simulink model "rocket_6dof_simulation"  (R2026b)
settings: Solver=ode4  StopTime=sim_stopTime  FixedStep=sim_fixedStep
undefined symbols (not defined in the file): aero_refLength, CG, chute_attachBody, chute_CdS, chute_inflateTau, chute_riserLength, Cl_delta, Cl_p, Cm_a, Cm_q, Cn_b, Cn_r, command_stepTime, controller_inner_Kp, controller_outer_Kp, controller_outer_maxRateCmd, CP, Cx_0, Cy_0, Cy_b, Cz_0, Cz_a, environment_g, environment_wind, fin_actuatorTau, fin_maxDeflection, fin_maxRate, Fth, initial_euler, initial_position, initial_pqr, initial_velocityBody, Isp, propulsion_cutoffTime, rocket_cg0, rocket_mass0, rocket_massDry, sensor_attitudeTau, sensor_gyroTau
libraries: aerolibasang x3, simulink x3, aerolibatmos2 x1, shared6dof x1
settings Model: Creator=kiwamoto  LastModifiedBy=kiwamoto

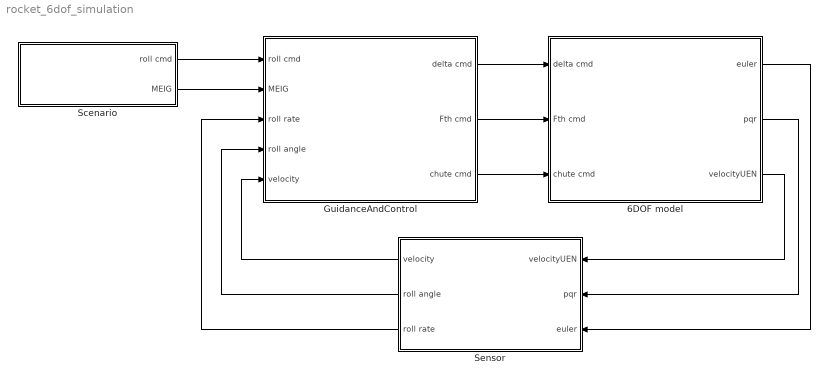
== system rocket_6dof_simulation ==
  6DOF model : Subsystem
  GuidanceAndControl : Subsystem
  Scenario : Subsystem
  Sensor : Subsystem
  wires:
  Scenario/1(roll cmd) -> GuidanceAndControl/1(roll cmd)
  GuidanceAndControl/1(delta cmd) -> 6DOF model/1(delta cmd)
  6DOF model/2(pqr) -> Sensor/2(pqr)
  6DOF model/1(euler) -> Sensor/3(euler)
  Sensor/2(roll angle) -> GuidanceAndControl/4(roll angle)
  Sensor/3(roll rate) -> GuidanceAndControl/3(roll rate)
  GuidanceAndControl/2(Fth cmd) -> 6DOF model/2(Fth cmd)
  Scenario/2(MEIG) -> GuidanceAndControl/2(MEIG)
  6DOF model/3(velocityUEN) -> Sensor/1(velocityUEN)
  GuidanceAndControl/3(chute cmd) -> 6DOF model/3(chute cmd)
  Sensor/1(velocity) -> GuidanceAndControl/5(velocity)

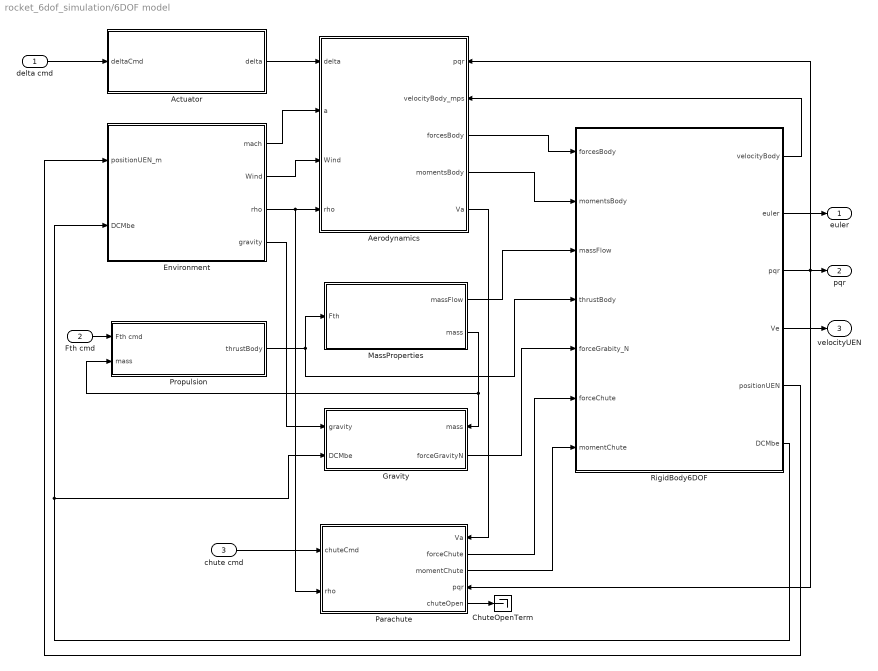
== system rocket_6dof_simulation/6DOF model ==
  delta cmd : Inport
  Fth cmd : Inport  Port=2
  chute cmd : Inport  Port=3
  Actuator : Subsystem
  Aerodynamics : Subsystem
      settings: PortSchema="{\"entries\":[{\"content\":{\"sides\":[{\"content\":{\"connectorIds\":[\"In1\",\"In2\",\"In3\",\"In4\"]},\"type\":\"ConnectorPlacement.EquallySpacedRectSide\",\"uuid\":\"af4c3f3a-b32b-4852-bfef-16d4a55bc85d\"},{\"content\":{\"connectorIds\":[\"In5\",\"In6\",\"Out1\",\"Out2\",\"Out3\"],\"side\":\"RIGHT\"},\"type\":\"ConnectorPlacement.EquallySpacedRectSide\",\"uuid\":\"ec426dca-c226-4b80-bf23-7134222deebc\"},{\"content\":{\"side\":\"TOP\"},\"type\":\"ConnectorPlacement.EquallySpacedRectSide\",\"uuid\":\"6bf281c2-d4c8-4f95-a415-10d5fcb30e4a\"}]},\"type\":\"ConnectorPlacement.EquallySpacedConnector\",\"uuid\":\"b5802e10-4233-47a2-b97a-a8820a58bc73\"}],\"packageUris\":[\"http://schema.mathworks.com/mf0/Connector/R2020b\"],\"version\":\"1.0\"}"
  ChuteOpenTerm : Terminator
  Environment : Subsystem
  Gravity : Subsystem
      settings: PortSchema="{\"entries\":[{\"content\":{\"sides\":[{\"content\":{\"connectorIds\":[\"In1\",\"In2\"]},\"type\":\"ConnectorPlacement.EquallySpacedRectSide\",\"uuid\":\"58b48f2a-cd32-4d34-a1ae-ee392d32123b\"},{\"content\":{\"connectorIds\":[\"In3\",\"Out1\"],\"side\":\"RIGHT\"},\"type\":\"ConnectorPlacement.EquallySpacedRectSide\",\"uuid\":\"b043d20d-e312-4365-ac79-6f9f081e3e75\"},{\"content\":{\"side\":\"TOP\"},\"type\":\"ConnectorPlacement.EquallySpacedRectSide\",\"uuid\":\"7786ccd6-2d55-46d0-949f-224f2e6bbbde\"}]},\"type\":\"ConnectorPlacement.EquallySpacedConnector\",\"uuid\":\"7e0c739f-134e-4285-a217-42daec375290\"}],\"packageUris\":[\"http://schema.mathworks.com/mf0/Connector/R2020b\"],\"version\":\"1.0\"}"
  MassProperties : Subsystem
  Parachute : Subsystem
      settings: PortSchema="{\"entries\":[{\"content\":{\"sides\":[{\"content\":{\"connectorIds\":[\"In1\",\"In2\"]},\"type\":\"ConnectorPlacement.EquallySpacedRectSide\",\"uuid\":\"ab562e91-55ed-4f52-87b8-211519146483\"},{\"content\":{\"connectorIds\":[\"In3\",\"Out1\",\"Out2\",\"In4\",\"Out3\"],\"side\":\"RIGHT\"},\"type\":\"ConnectorPlacement.EquallySpacedRectSide\",\"uuid\":\"d1f95e4e-60be-4e36-afec-0b6bd2c0f004\"},{\"content\":{\"side\":\"TOP\"},\"type\":\"ConnectorPlacement.EquallySpacedRectSide\",\"uuid\":\"dc12724e-5caf-4014-9240-a32a59dbf896\"}]},\"type\":\"ConnectorPlacement.EquallySpacedConnector\",\"uuid\":\"e57dcaa1-2a9c-4da6-8406-b82df234227e\"}],\"packageUris\":[\"http://schema.mathworks.com/mf0/Connector/R2020b\"],\"version\":\"1.0\"}"
  Propulsion : Subsystem
  RigidBody6DOF : Subsystem
  euler : Outport
  pqr : Outport  Port=2
  velocityUEN : Outport  Port=3
  wires:
  RigidBody6DOF/3(pqr) -> Parachute/4(pqr), pqr/1, Aerodynamics/5(pqr)
  MassProperties/2(mass) -> Propulsion/2(mass), Gravity/3(mass)
  RigidBody6DOF/1(velocityBody) -> Aerodynamics/6(velocityBody_mps)
  Actuator/1(delta) -> Aerodynamics/1(delta)
  Aerodynamics/2(momentsBody) -> RigidBody6DOF/2(momentsBody)
  Aerodynamics/1(forcesBody) -> RigidBody6DOF/1(forcesBody)
  Propulsion/1(thrustBody) -> RigidBody6DOF/4(thrustBody), MassProperties/1(Fth)
  delta cmd/1 -> Actuator/1(deltaCmd)
  RigidBody6DOF/2(euler) -> euler/1
  Environment/3(rho) -> Aerodynamics/4(rho), Parachute/2(rho)
  Environment/4(gravity) -> Gravity/1(gravity)
  RigidBody6DOF/6(DCMbe) -> Gravity/2(DCMbe), Environment/2(DCMbe)
  Gravity/1(forceGravityN) -> RigidBody6DOF/5(forceGrabity_N)
  Environment/2(Wind) -> Aerodynamics/3(Wind)
  Environment/1(mach) -> Aerodynamics/2(a)
  RigidBody6DOF/5(positionUEN) -> Environment/1(positionUEN_m)
  Fth cmd/1 -> Propulsion/1(Fth cmd)
  MassProperties/1(massFlow) -> RigidBody6DOF/3(massFlow)
  chute cmd/1 -> Parachute/1(chuteCmd)
  Aerodynamics/3(Va) -> Parachute/3(Va)
  Parachute/3(chuteOpen) -> ChuteOpenTerm/1
  Parachute/1(forceChute) -> RigidBody6DOF/6(forceChute)
  Parachute/2(momentChute) -> RigidBody6DOF/7(momentChute)
  RigidBody6DOF/4(Ve) -> velocityUEN/1

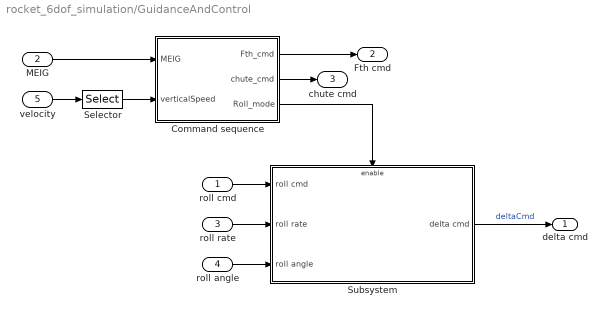
== system rocket_6dof_simulation/GuidanceAndControl ==
  roll cmd : Inport
  MEIG : Inport  Port=2
  roll rate : Inport  Port=3
  roll angle : Inport  Port=4
  velocity : Inport  Port=5
  Command sequence : Stateflow chart  TreatAsAtomicUnit=on
      settings: PortSchema="{\"entries\":[{\"content\":{\"sides\":[{\"content\":{\"connectorIds\":[\"In1\",\"In2\"]},\"type\":\"ConnectorPlacement.EquallySpacedRectSide\",\"uuid\":\"95c67331-47e3-44af-bd01-16a94959fc95\"},{\"content\":{\"connectorIds\":[\"Out1\",\"Out3\",\"Out2\"],\"side\":\"RIGHT\"},\"type\":\"ConnectorPlacement.EquallySpacedRectSide\",\"uuid\":\"42b891d2-3784-42c1-a532-d1c942f19e32\"},{\"content\":{\"side\":\"TOP\"},\"type\":\"ConnectorPlacement.EquallySpacedRectSide\",\"uuid\":\"6230014a-0262-43f4-a38a-a38e632e5bb9\"}]},\"type\":\"ConnectorPlacement.EquallySpacedConnector\",\"uuid\":\"a3f4a931-66e7-452b-9163-9591630e354f\"}],\"packageUris\":[\"http://schema.mathworks.com/mf0/Connector/R2020b\"],\"version\":\"1.0\"}"
  Selector : Selector  InputPortWidth=3  IndexOptions=Index vector (dialog)  Indices=1  OutputSizes=1  RuntimeRangeChecks=off
  Subsystem : Subsystem
  delta cmd : Outport
  Fth cmd : Outport  Port=2
  chute cmd : Outport  Port=3
  wires:
  Command sequence/1(Fth_cmd) -> Fth cmd/1
  MEIG/1 -> Command sequence/1(MEIG)
  roll cmd/1 -> Subsystem/1(roll cmd)
  roll rate/1 -> Subsystem/2(roll rate)
  roll angle/1 -> Subsystem/3(roll angle)
  Subsystem/1(delta cmd) -> delta cmd/1  "deltaCmd"
  Command sequence/2(Roll_mode) -> Subsystem/Enable
  velocity/1 -> Selector/1
  Command sequence/3(chute_cmd) -> chute cmd/1
  Selector/1 -> Command sequence/2(verticalSpeed)

== system rocket_6dof_simulation/Scenario ==
  On : Constant
  RollCommandStep : Step  Time=command_stepTime  FinalValue=command_rollStep  SampleTime=0
  roll cmd : Outport
  MEIG : Outport  Port=2
  wires:
  RollCommandStep/1 -> roll cmd/1  "phiCmd"
  On/1 -> MEIG/1

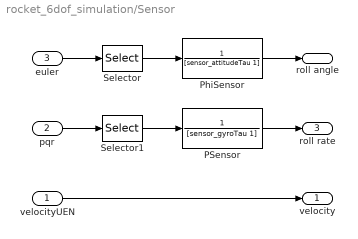
== system rocket_6dof_simulation/Sensor ==
  velocityUEN : Inport
  pqr : Inport  Port=2
  euler : Inport  Port=3
  PSensor : TransferFcn  Denominator=[sensor_gyroTau 1]
  PhiSensor : TransferFcn  Denominator=[sensor_attitudeTau 1]
  Selector : Selector  InputPortWidth=3  IndexOptions=Index vector (dialog)  Indices=1  OutputSizes=1  RuntimeRangeChecks=off
  Selector1 : Selector  InputPortWidth=3  IndexOptions=Index vector (dialog)  Indices=1  OutputSizes=1  RuntimeRangeChecks=off
  velocity : Outport
  roll angle : Outport  Port=2
  roll rate : Outport  Port=3
  wires:
  pqr/1 -> Selector1/1
  PhiSensor/1 -> roll angle/1
  Selector/1 -> PhiSensor/1
  Selector1/1 -> PSensor/1
  euler/1 -> Selector/1
  PSensor/1 -> roll rate/1
  velocityUEN/1 -> velocity/1

== system rocket_6dof_simulation/6DOF model/Actuator ==
  deltaCmd : Inport
  FinActuator : TransferFcn  Denominator=[fin_actuatorTau 1]
  FinRateLimiter : RateLimiter  RisingSlewLimit=fin_maxRate  FallingSlewLimit=-fin_maxRate  SampleTimeMode=inherited
  FinSaturation : Saturate  UpperLimit=fin_maxDeflection  LowerLimit=-fin_maxDeflection
  delta : Outport
  wires:
  deltaCmd/1 -> FinRateLimiter/1
  FinRateLimiter/1 -> FinSaturation/1
  FinSaturation/1 -> FinActuator/1
  FinActuator/1 -> delta/1  "delta"

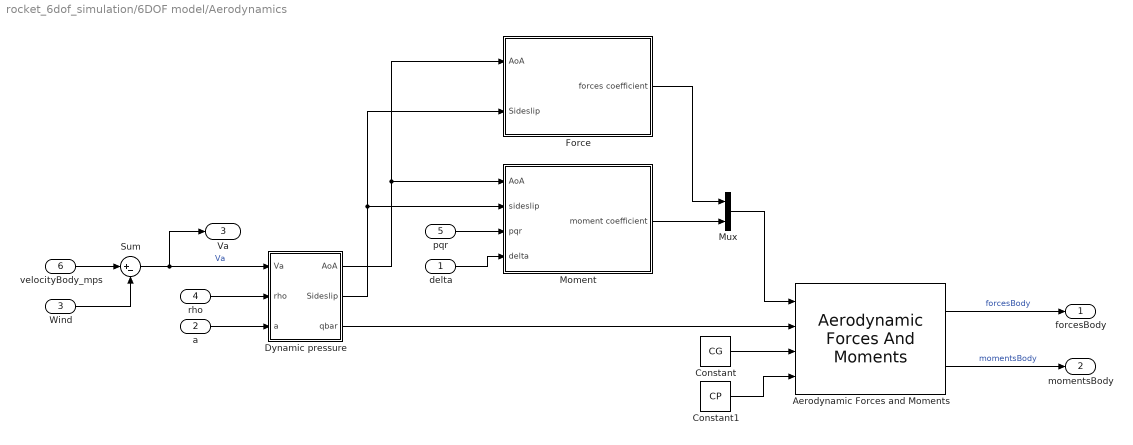
== system rocket_6dof_simulation/6DOF model/Aerodynamics ==
  delta : Inport
  a : Inport  Port=2
  Wind : Inport  Port=3
  rho : Inport  Port=4
  pqr : Inport  Port=5
  velocityBody_mps : Inport  Port=6
  "Aerodynamic Forces and Moments " : AerodynamicForcesAndMoments  S=aero_refArea  b=aero_refLength  cbar=aero_refLength
  Constant : Constant  Value=CG
  Constant1 : Constant  Value=CP
  Dynamic pressure : Subsystem
  Force : Subsystem
  Moment : Subsystem
  Mux : Mux  Inputs=2
  Sum : Sum  Inputs=|+-
  forcesBody : Outport
  momentsBody : Outport  Port=2
  Va : Outport  Port=3
  wires:
  delta/1 -> Moment/4(delta)
  rho/1 -> Dynamic pressure/2(rho)
  velocityBody_mps/1 -> Sum/1
  Wind/1 -> Sum/2
  Sum/1 -> Dynamic pressure/1(Va), Va/1  "Va"
  a/1 -> Dynamic pressure/3(a)
  "Aerodynamic Forces and Moments "/1 -> forcesBody/1  "forcesBody"
  "Aerodynamic Forces and Moments "/2 -> momentsBody/1  "momentsBody"
  Dynamic pressure/3(qbar) -> "Aerodynamic Forces and Moments "/2
  pqr/1 -> Moment/3(pqr)
  Mux/1 -> "Aerodynamic Forces and Moments "/1
  Moment/1(moment coefficient) -> Mux/2
  Force/1(forces coefficient) -> Mux/1
  Dynamic pressure/1(AoA) -> Force/1(AoA), Moment/1(AoA)
  Dynamic pressure/2(Sideslip) -> Force/2(Sideslip), Moment/2(sideslip)
  Constant/1 -> "Aerodynamic Forces and Moments "/3
  Constant1/1 -> "Aerodynamic Forces and Moments "/4

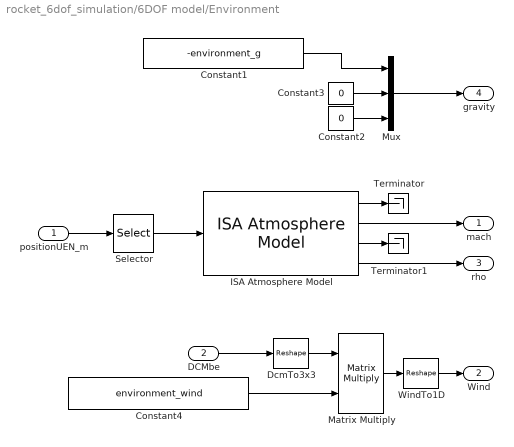
== system rocket_6dof_simulation/6DOF model/Environment ==
  positionUEN_m : Inport
  DCMbe : Inport  Port=2
  Constant1 : Constant  Value=-environment_g
  Constant2 : Constant  Value=0
  Constant3 : Constant  Value=0
  Constant4 : Constant  Value=environment_wind
  DcmTo3x3 : Reshape  OutputDimensionality=Customize  OutputDimensions=[3 3]
  ISA Atmosphere Model : aerolibatmos2/ISA Atmosphere Model  useExtended=off  action=None  custom=off  viscosityOut=off  g=9.80665  gamma=1.4  R=287.0531  L=0.0065  h_trop=11000  h_strat=20000  rho0=1.225  P0=101325  T0=288.15  h0=0  S=110.4  Tref=273.15  muref=1.716e-5
  Matrix Multiply : Product  Multiplication=Matrix(*)
  Mux : Mux  Inputs=3
  Selector : Selector  InputPortWidth=3  IndexOptions=Index vector (dialog)  Indices=1  OutputSizes=1  RuntimeRangeChecks=off
  Terminator : Terminator
  Terminator1 : Terminator
  WindTo1D : Reshape
  mach : Outport
  Wind : Outport  Port=2
  rho : Outport  Port=3
  gravity : Outport  Port=4
  wires:
  ISA Atmosphere Model/4 -> rho/1
  Mux/1 -> gravity/1
  Constant2/1 -> Mux/3
  Constant3/1 -> Mux/2
  Constant1/1 -> Mux/1
  Constant4/1 -> Matrix Multiply/2
  ISA Atmosphere Model/2 -> mach/1
  ISA Atmosphere Model/1 -> Terminator/1
  ISA Atmosphere Model/3 -> Terminator1/1
  positionUEN_m/1 -> Selector/1
  Selector/1 -> ISA Atmosphere Model/1
  Matrix Multiply/1 -> WindTo1D/1
  WindTo1D/1 -> Wind/1
  DCMbe/1 -> DcmTo3x3/1
  DcmTo3x3/1 -> Matrix Multiply/1

== system rocket_6dof_simulation/6DOF model/Gravity ==
  gravity : Inport
  DCMbe : Inport  Port=2
  mass : Inport  Port=3
  DcmTo3x3 : Reshape  OutputDimensionality=Customize  OutputDimensions=[3 3]
  GravityTo1D : Reshape
  Product : Product  Multiplication=Matrix(*)
  Product1 : Product
  forceGravityN : Outport
  wires:
  Product/1 -> GravityTo1D/1
  GravityTo1D/1 -> forceGravityN/1
  DCMbe/1 -> DcmTo3x3/1
  DcmTo3x3/1 -> Product/1
  gravity/1 -> Product1/1
  mass/1 -> Product1/2
  Product1/1 -> Product/2

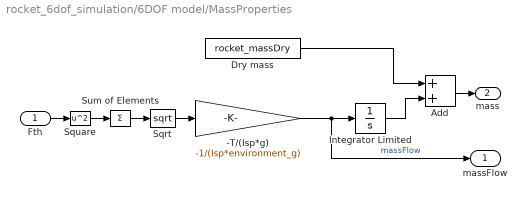
== system rocket_6dof_simulation/6DOF model/MassProperties ==
  Fth : Inport
  -T/(Isp*g) : Gain  Gain=-1/(Isp*environment_g)
  Add : Sum
  Dry mass : Constant  Value=rocket_massDry
  Integrator Limited : Integrator  InitialCondition=rocket_mass0 - rocket_massDry  LimitOutput=on  UpperSaturationLimit=rocket_mass0 - rocket_massDry  LowerSaturationLimit=0
  Sqrt : Sqrt
  Square : Math  Operator=square
  Sum of Elements : Sum  Inputs=+
  massFlow : Outport
  mass : Outport  Port=2
  wires:
  Dry mass/1 -> Add/1
  Integrator Limited/1 -> Add/2
  Add/1 -> mass/1
  -T/(Isp*g)/1 -> Integrator Limited/1, massFlow/1  "massFlow"
  Fth/1 -> Square/1
  Square/1 -> Sum of Elements/1
  Sum of Elements/1 -> Sqrt/1
  Sqrt/1 -> -T/(Isp*g)/1

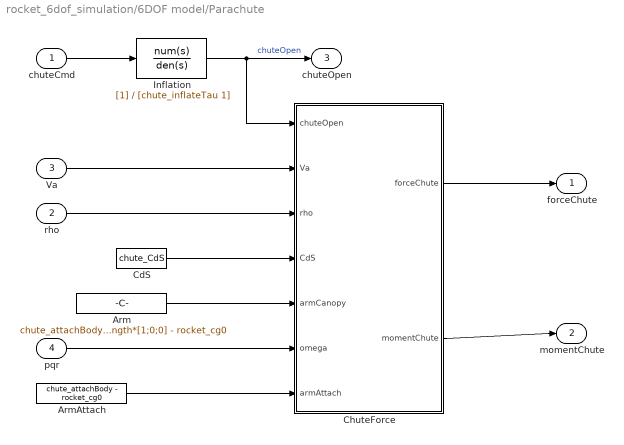
== system rocket_6dof_simulation/6DOF model/Parachute ==
  chuteCmd : Inport
  rho : Inport  Port=2
  Va : Inport  Port=3
  pqr : Inport  Port=4
  Arm : Constant  Value=chute_attachBody + chute_riserLength*[1;0;0] - rocket_cg0
  ArmAttach : Constant  Value=chute_attachBody - rocket_cg0
  CdS : Constant  Value=chute_CdS
  ChuteForce : MATLAB Function  TreatAsAtomicUnit=on
  Inflation : TransferFcn  Denominator=[chute_inflateTau 1]
  forceChute : Outport
  momentChute : Outport  Port=2
  chuteOpen : Outport  Port=3
  wires:
  chuteCmd/1 -> Inflation/1
  Inflation/1 -> ChuteForce/1(chuteOpen), chuteOpen/1  "chuteOpen"
  Va/1 -> ChuteForce/2(Va)
  rho/1 -> ChuteForce/3(rho)
  CdS/1 -> ChuteForce/4(CdS)
  Arm/1 -> ChuteForce/5(armCanopy)
  ChuteForce/1(forceChute) -> forceChute/1
  ChuteForce/2(momentChute) -> momentChute/1
  pqr/1 -> ChuteForce/6(omega)
  ArmAttach/1 -> ChuteForce/7(armAttach)

== system rocket_6dof_simulation/6DOF model/Propulsion ==
  Fth cmd : Inport
  mass : Inport  Port=2
  Compare To Constant : simulink/Logic and Bit Operations/Compare To Constant  relop=>  const=rocket_massDry  OutDataTypeStr=boolean
  Product : Product
  ThrustMux : Mux  Inputs=3
  ZeroY : Constant  Value=0
  ZeroZ : Constant  Value=0
  burn delay : TransferFcn  Denominator=[0.05 1]
  thrustBody : Outport
  wires:
  ZeroY/1 -> ThrustMux/2
  ZeroZ/1 -> ThrustMux/3
  ThrustMux/1 -> thrustBody/1
  Fth cmd/1 -> burn delay/1
  mass/1 -> Compare To Constant/1
  Product/1 -> ThrustMux/1  "thrust"
  Compare To Constant/1 -> Product/1
  burn delay/1 -> Product/2

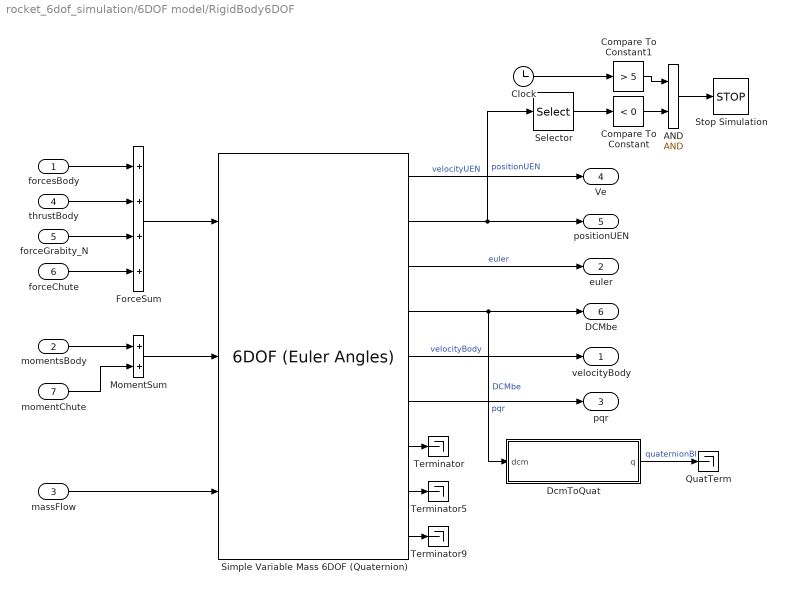
== system rocket_6dof_simulation/6DOF model/RigidBody6DOF ==
  forcesBody : Inport
  momentsBody : Inport  Port=2
  massFlow : Inport  Port=3
  thrustBody : Inport  Port=4
  forceGrabity_N : Inport  Port=5
  forceChute : Inport  Port=6
  momentChute : Inport  Port=7
  AND : Logic  IconShape=distinctive  AllPortsSameDT=off  OutDataTypeStr=boolean
  Clock : Clock
  Compare To Constant : simulink/Logic and Bit Operations/Compare To Constant  relop=<  const=0  OutDataTypeStr=boolean
  Compare To Constant1 : simulink/Logic and Bit Operations/Compare To Constant  relop=>  const=5  OutDataTypeStr=boolean
  DcmToQuat : MATLAB Function  TreatAsAtomicUnit=on
  ForceSum : Sum  Inputs=++++
  MomentSum : Sum
  QuatTerm : Terminator
  Selector : Selector  InputPortWidth=3  IndexOptions=Index vector (dialog)  Indices=1  OutputSizes=1  RuntimeRangeChecks=off
  Simple Variable Mass 6DOF (Quaternion) : shared6dof/6DOF (Euler Angles)  units=Metric (MKS)  mtype=Simple Variable  rep=Quaternion  xme_0=initial_position(:).'  Vm_0=initial_velocityBody(:).'  eul_0=initial_euler(:).'  pm_0=initial_pqr(:).'  mass_0=rocket_mass0  mass_e=rocket_massDry  mass_f=rocket_mass0  inertia=eye(3)  inertia_e=rocket_inertiaDry  inertia_f=rocket_inertia0  k_quat=1.0  vre_flag=off  abi_flag=off  aMode=aMode  xme_statename=''  Vm_statename=''  eul_statename=''  quat_statename=''  pm_statename=''  mass_statename=''
  Stop Simulation : Stop
  Terminator : Terminator
  Terminator5 : Terminator
  Terminator9 : Terminator
  velocityBody : Outport
  euler : Outport  Port=2
  pqr : Outport  Port=3
  Ve : Outport  Port=4
  positionUEN : Outport  Port=5
  DCMbe : Outport  Port=6
  wires:
  forcesBody/1 -> ForceSum/1
  thrustBody/1 -> ForceSum/2
  forceGrabity_N/1 -> ForceSum/3
  ForceSum/1 -> Simple Variable Mass 6DOF (Quaternion)/1
  Simple Variable Mass 6DOF (Quaternion)/2 -> Selector/1, positionUEN/1  "positionUEN"
  Simple Variable Mass 6DOF (Quaternion)/3 -> euler/1  "euler"
  Simple Variable Mass 6DOF (Quaternion)/4 -> DCMbe/1, DcmToQuat/1(dcm)  "DCMbe"
  Simple Variable Mass 6DOF (Quaternion)/5 -> velocityBody/1  "velocityBody"
  Simple Variable Mass 6DOF (Quaternion)/6 -> pqr/1  "pqr"
  Simple Variable Mass 6DOF (Quaternion)/7 -> Terminator/1
  Simple Variable Mass 6DOF (Quaternion)/8 -> Terminator5/1
  Simple Variable Mass 6DOF (Quaternion)/9 -> Terminator9/1
  DcmToQuat/1(q) -> QuatTerm/1  "quaternionBI"
  massFlow/1 -> Simple Variable Mass 6DOF (Quaternion)/3
  Selector/1 -> Compare To Constant/1
  Compare To Constant/1 -> AND/2
  AND/1 -> Stop Simulation/1
  Compare To Constant1/1 -> AND/1
  Clock/1 -> Compare To Constant1/1
  Simple Variable Mass 6DOF (Quaternion)/1 -> Ve/1  "velocityUEN"
  forceChute/1 -> ForceSum/4
  momentsBody/1 -> MomentSum/1
  momentChute/1 -> MomentSum/2
  MomentSum/1 -> Simple Variable Mass 6DOF (Quaternion)/2

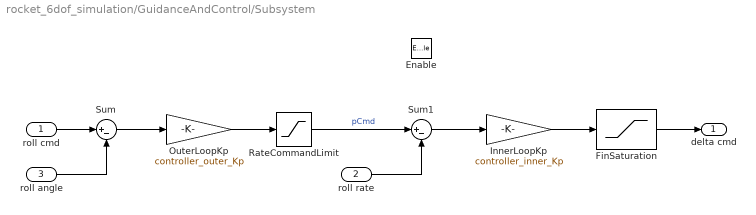
== system rocket_6dof_simulation/GuidanceAndControl/Subsystem ==
  roll cmd : Inport
  roll rate : Inport  Port=2
  roll angle : Inport  Port=3
  Enable : EnablePort  StatesWhenEnabling=reset
  FinSaturation : Saturate  UpperLimit=fin_maxDeflection  LowerLimit=-fin_maxDeflection
  InnerLoopKp : Gain  Gain=controller_inner_Kp
  OuterLoopKp : Gain  Gain=controller_outer_Kp
  RateCommandLimit : Saturate  UpperLimit=controller_outer_maxRateCmd  LowerLimit=-controller_outer_maxRateCmd
  Sum : Sum  Inputs=|+-
  Sum1 : Sum  Inputs=|+-
  delta cmd : Outport  OutputWhenDisabled=reset  InitialOutput=[0]
  wires:
  roll rate/1 -> Sum1/2
  InnerLoopKp/1 -> FinSaturation/1
  Sum1/1 -> InnerLoopKp/1
  Sum/1 -> OuterLoopKp/1
  RateCommandLimit/1 -> Sum1/1  "pCmd"
  roll cmd/1 -> Sum/1
  OuterLoopKp/1 -> RateCommandLimit/1
  roll angle/1 -> Sum/2
  FinSaturation/1 -> delta cmd/1

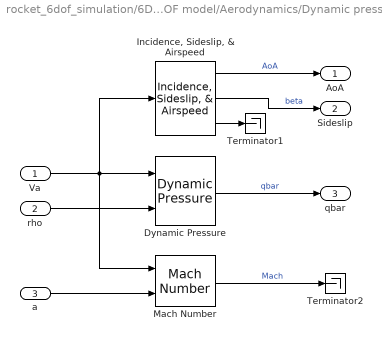
== system rocket_6dof_simulation/6DOF model/Aerodynamics/Dynamic pressure ==
  Va : Inport
  rho : Inport  Port=2
  a : Inport  Port=3
  Dynamic Pressure : aerolibasang/Dynamic Pressure
  "Incidence, Sideslip, & Airspeed" : aerolibasang/Incidence, Sideslip, & Airspeed
  Mach Number : aerolibasang/Mach Number
  Terminator1 : Terminator
  Terminator2 : Terminator
  AoA : Outport
  Sideslip : Outport  Port=2
  qbar : Outport  Port=3
  wires:
  Dynamic Pressure/1 -> qbar/1  "qbar"
  Mach Number/1 -> Terminator2/1  "Mach"
  rho/1 -> Dynamic Pressure/2
  a/1 -> Mach Number/2
  Va/1 -> "Incidence, Sideslip, & Airspeed"/1, Mach Number/1, Dynamic Pressure/1
  "Incidence, Sideslip, & Airspeed"/1 -> AoA/1  "AoA"
  "Incidence, Sideslip, & Airspeed"/2 -> Sideslip/1  "beta"
  "Incidence, Sideslip, & Airspeed"/3 -> Terminator1/1

== system rocket_6dof_simulation/6DOF model/Aerodynamics/Force ==
  AoA : Inport
  Sideslip : Inport  Port=2
  Coeffs : Constant  Value=[Cx_0; Cy_0; Cz_0; Cy_b; Cz_a]
  ForceCoefficients : MATLAB Function  TreatAsAtomicUnit=on
  To1D : Reshape
  forces coefficient : Outport
  wires:
  AoA/1 -> ForceCoefficients/1(alpha)
  Sideslip/1 -> ForceCoefficients/2(beta)
  Coeffs/1 -> ForceCoefficients/3(coeffs)
  ForceCoefficients/1(C) -> To1D/1
  To1D/1 -> forces coefficient/1

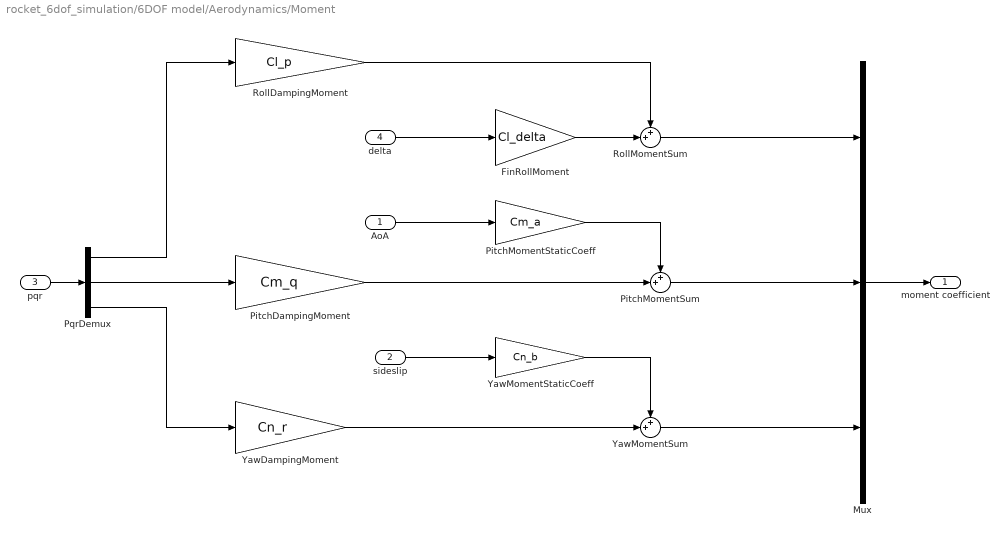
== system rocket_6dof_simulation/6DOF model/Aerodynamics/Moment ==
  AoA : Inport
  sideslip : Inport  Port=2
  pqr : Inport  Port=3
  delta : Inport  Port=4
  FinRollMoment : Gain  Gain=Cl_delta
  Mux : Mux  Inputs=3
  PitchDampingMoment : Gain  Gain=Cm_q
  PitchMomentStaticCoeff : Gain  Gain=Cm_a
  PitchMomentSum : Sum  Inputs=++|
  PqrDemux : Demux  Outputs=3
  RollDampingMoment : Gain  Gain=Cl_p
  RollMomentSum : Sum  Inputs=++|
  YawDampingMoment : Gain  Gain=Cn_r
  YawMomentStaticCoeff : Gain  Gain=Cn_b
  YawMomentSum : Sum  Inputs=++|
  moment coefficient : Outport
  wires:
  sideslip/1 -> YawMomentStaticCoeff/1
  FinRollMoment/1 -> RollMomentSum/2
  PqrDemux/3 -> YawDampingMoment/1
  PqrDemux/1 -> RollDampingMoment/1
  PqrDemux/2 -> PitchDampingMoment/1
  pqr/1 -> PqrDemux/1
  delta/1 -> FinRollMoment/1
  AoA/1 -> PitchMomentStaticCoeff/1
  Mux/1 -> moment coefficient/1
  YawMomentSum/1 -> Mux/3
  PitchMomentSum/1 -> Mux/2
  RollDampingMoment/1 -> RollMomentSum/1
  RollMomentSum/1 -> Mux/1
  PitchDampingMoment/1 -> PitchMomentSum/2
  YawDampingMoment/1 -> YawMomentSum/2
  PitchMomentStaticCoeff/1 -> PitchMomentSum/1
  YawMomentStaticCoeff/1 -> YawMomentSum/1

== matlab function rocket_6dof_simulation/6DOF model/Parachute/ChuteForce ==
  data: chuteOpen input; forceChute output; Va input; rho input; CdS input; armCanopy input; momentChute output; omega input; armAttach input
function [forceChute, momentChute] = chute_force(chuteOpen, Va, rho, CdS, armCanopy, omega, armAttach)
%#codegen
% Parachute forces and moments on the vehicle (body frame).
%
%   armCanopy : Canopy center - CG [m]; location used to evaluate drag.
%   armAttach : Attachment point - CG [m]; location where force enters the body.
%
% Distinguish the two positions. Drag magnitude and direction are set at the canopy,
% but the riser transmits force at the attachment, which defines the moment arm.
% Using canopy position for both overestimates restoring stiffness by the arm ratio.
%
% Risers transmit tension only. Drag opposes the relative air velocity, pulling
% the vehicle toward the canopy, so this formulation represents tension-only loading.

canopy = armCanopy(:);
attach = armAttach(:);

% Air-relative velocity at the canopy; lateral motion due to body rotation produces damping.
vCanopy = Va(:) + cross(omega(:), canopy);
speed   = norm(vCanopy);

forceChute  = -0.5 * rho * speed * vCanopy * CdS * chuteOpen;
momentChute = cross(attach, forceChute);
end

== matlab function rocket_6dof_simulation/6DOF model/RigidBody6DOF/DcmToQuat ==
  data: dcm input; q output
function q = quaternion_from_dcm(dcm)
%#codegen
% Construct quaternion [q0 q1 q2 q3] from DCMbe (body <- UEN).
% The convention quat2dcm(q) = dcm matches the default interpretation in animate_flight.
% Compute explicitly instead of using dcm2quat to make Simulink size inference deterministic.
q = zeros(1, 4);
tr = dcm(1,1) + dcm(2,2) + dcm(3,3);
if tr > 0
    s = sqrt(tr + 1) * 2;
    q(1) = 0.25 * s;
    q(2) = (dcm(2,3) - dcm(3,2)) / s;
    q(3) = (dcm(3,1) - dcm(1,3)) / s;
    q(4) = (dcm(1,2) - dcm(2,1)) / s;
elseif dcm(1,1) > dcm(2,2) && dcm(1,1) > dcm(3,3)
    s = sqrt(1 + dcm(1,1) - dcm(2,2) - dcm(3,3)) * 2;
    q(1) = (dcm(2,3) - dcm(3,2)) / s;
    q(2) = 0.25 * s;
    q(3) = (dcm(1,2) + dcm(2,1)) / s;
    q(4) = (dcm(3,1) + dcm(1,3)) / s;
elseif dcm(2,2) > dcm(3,3)
    s = sqrt(1 + dcm(2,2) - dcm(1,1) - dcm(3,3)) * 2;
    q(1) = (dcm(3,1) - dcm(1,3)) / s;
    q(2) = (dcm(1,2) + dcm(2,1)) / s;
    q(3) = 0.25 * s;
    q(4) = (dcm(2,3) + dcm(3,2)) / s;
else
    s = sqrt(1 + dcm(3,3) - dcm(1,1) - dcm(2,2)) * 2;
    q(1) = (dcm(1,2) - dcm(2,1)) / s;
    q(2) = (dcm(3,1) + dcm(1,3)) / s;
    q(3) = (dcm(2,3) + dcm(3,2)) / s;
    q(4) = 0.25 * s;
end
q = q / norm(q);
if q(1) < 0
    q = -q;
end
end

== stateflow chart rocket_6dof_simulation/GuidanceAndControl/Command sequence ==
  state Standby
    Fth_cmd = 0;
    Roll_mode = 0;
    chute_cmd = 0;
  state Launch
    state Ingition
      Fth_cmd = Fth;
    state Roll_control
      Roll_mode = 1;
    Ingition -> Roll_control : [after(1,'sec')]
  state MECO
    Fth_cmd = 0;
    Roll_mode = 0;
  state Recovery
    chute_cmd = 1;
  (default) -> Standby
  Standby -> Ingition : [MEIG]
  Launch -> MECO : [after(propulsion_cutoffTime,'sec')]
  MECO -> Recovery : [verticalSpeed <= 0]
  data: Fth parameter; Fth_cmd output; MEIG input; propulsion_cutoffTime parameter; Roll_mode output; verticalSpeed input; chute_cmd output

== matlab function rocket_6dof_simulation/6DOF model/Aerodynamics/Force/ForceCoefficients ==
  data: alpha input; C output; beta input; coeffs input
function C = force_coefficients(alpha, beta, coeffs)
%#codegen
% Body-axis aerodynamic force coefficients [Cx; Cy; Cz].
%
%   alpha, beta : Angle of attack and sideslip angle [rad]
%   coeffs      : [Cx_0; Cy_0; Cz_0; Cy_b; Cz_a]
%
%   Axial force : Cx = Cx_0 * cos(alpha) * cos(beta)
%   Normal force: Cz = Cz_0 + Cz_a * sin(alpha) * cos(alpha)
%   Side force  : Analogous expression using beta

Cx_0 = coeffs(1);
Cy_0 = coeffs(2);
Cz_0 = coeffs(3);
Cy_b = coeffs(4);
Cz_a = coeffs(5);

Cx = Cx_0 * cos(alpha) * cos(beta);
Cy = Cy_0 + Cy_b * sin(beta)  * cos(beta);
Cz = Cz_0 + Cz_a * sin(alpha) * cos(alpha);

C = [Cx; Cy; Cz];
end
